simulink model "H04_ARM"  (R2026a)
settings: Solver=VariableStepAuto  MaxStep=tau/25
InitFcn:
  | tau = 1;
settings Model: Creator=Szalay  LastModifiedBy=Szalay

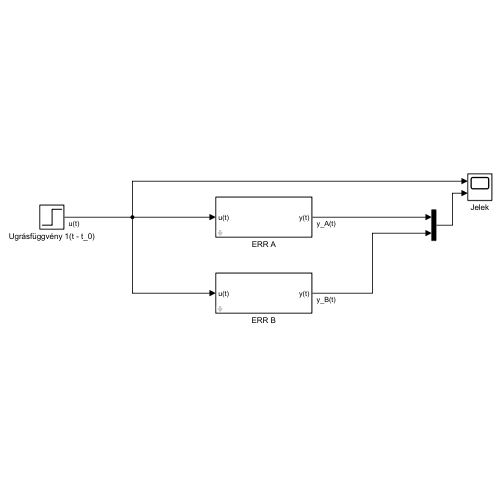
[thumbnail: Simulink's stored preview of the top-level diagram]
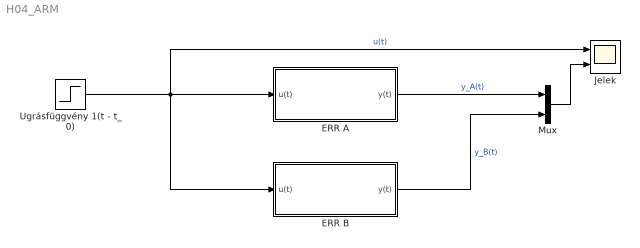
== system H04_ARM ==
  ERR A : Subsystem  mask(Elsőrendű rendszer){y_0=2.5, K=1, tau=tau}
      mask prompts: y_0 "A kimenet kezdeti értéke"; K "Állandult állapoti erősítés"; tau "Időállandó"
      mask help: A lineáris elsőrendű rendszer modellje.
      mask DialogControl ParameterGroupVar Prompt: Rendszerparaméterek
      mask DialogControl Container3 Prompt: Kezdeti érték
  ERR B : Subsystem  mask(Elsőrendű rendszer){y_0=-2.5, K=1, tau=tau}
      mask prompts: y_0 "A kimenet kezdeti értéke"; K "Állandult állapoti erősítés"; tau "Időállandó"
      mask help: A lineáris elsőrendű rendszer modellje.
      mask DialogControl ParameterGroupVar Prompt: Rendszerparaméterek
      mask DialogControl Container3 Prompt: Kezdeti érték
  Jelek : Scope  NumInputPorts=2
      settings: ActiveDisplayYMinimum=-3.125  ActiveDisplayYMaximum=3.125
  Mux : Mux  Inputs=2
  Ugrásfüggvény 1(t - t_0) : Step  Time=5  FinalValue=0.5  SampleTime=0
  wires:
  Mux/1 -> Jelek/2
  Ugrásfüggvény 1(t - t_0)/1 -> ERR B/1(u(t)), Jelek/1, ERR A/1(u(t))  "u(t)"
  ERR A/1(y(t)) -> Mux/1  "y_A(t)"
  ERR B/1(y(t)) -> Mux/2  "y_B(t)"

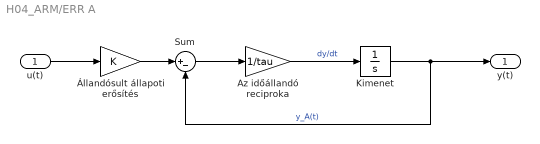
== system H04_ARM/ERR A ==
  u(t) : Inport
  Az időállandó reciproka : Gain  Gain=1/tau
  Kimenet : Integrator  InitialCondition=y_0
  Sum : Sum  Inputs=|+-
  Állandósult állapoti erősítés : Gain  Gain=K
  y(t) : Outport
  wires:
  u(t)/1 -> Állandósult állapoti erősítés/1
  Kimenet/1 -> y(t)/1, Sum/2  "y_A(t)"
  Az időállandó reciproka/1 -> Kimenet/1  "dy/dt"
  Sum/1 -> Az időállandó reciproka/1
  Állandósult állapoti erősítés/1 -> Sum/1

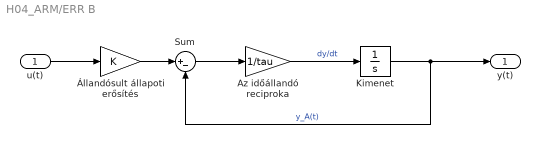
== system H04_ARM/ERR B ==
  u(t) : Inport
  Az időállandó reciproka : Gain  Gain=1/tau
  Kimenet : Integrator  InitialCondition=y_0
  Sum : Sum  Inputs=|+-
  Állandósult állapoti erősítés : Gain  Gain=K
  y(t) : Outport
  wires:
  Állandósult állapoti erősítés/1 -> Sum/1
  Sum/1 -> Az időállandó reciproka/1
  Az időállandó reciproka/1 -> Kimenet/1  "dy/dt"
  Kimenet/1 -> Sum/2, y(t)/1  "y_A(t)"
  u(t)/1 -> Állandósult állapoti erősítés/1
